simulink model "talos_navigation"  (R2023a)
settings: Solver=FixedStepDiscrete  StartTime=0.0  StopTime=10.0  FixedStep=1/1000.0  RelTol=1e-3  EnableMultiTasking=on
undefined symbols (not defined in the file): accel, child_frame_id, child_frame_id_SL_Info, data, data_SL_Info, header, layout, transform, transforms, transforms_SL_Info
libraries: ros2lib x187, simulink x9, sharedTrackingLibrary x1
(part 3 of 3)

== system talos_navigation/Parameters/estimator/process_noise_diag ==
  element_0 : ros2lib/Get Parameter  ParameterName=navigation__estimator__process_noise_diag_0  ParameterType=double  ParameterMaxArrayLength=16  ParameterInitialValue=5e-05  SampleTime=1/10.0  ModelName=ros2lib  BlockId=ParamGet_ros2lib_196
  element_1 : ros2lib/Get Parameter  ParameterName=navigation__estimator__process_noise_diag_1  ParameterType=double  ParameterMaxArrayLength=16  ParameterInitialValue=5e-05  SampleTime=1/10.0  ModelName=ros2lib  BlockId=ParamGet_ros2lib_196
  element_10 : ros2lib/Get Parameter  ParameterName=navigation__estimator__process_noise_diag_10  ParameterType=double  ParameterMaxArrayLength=16  ParameterInitialValue=0.0003  SampleTime=1/10.0  ModelName=ros2lib  BlockId=ParamGet_ros2lib_196
  element_11 : ros2lib/Get Parameter  ParameterName=navigation__estimator__process_noise_diag_11  ParameterType=double  ParameterMaxArrayLength=16  ParameterInitialValue=0.0003  SampleTime=1/10.0  ModelName=ros2lib  BlockId=ParamGet_ros2lib_196
  element_12 : ros2lib/Get Parameter  ParameterName=navigation__estimator__process_noise_diag_12  ParameterType=double  ParameterMaxArrayLength=16  ParameterInitialValue=0.0006  SampleTime=1/10.0  ModelName=ros2lib  BlockId=ParamGet_ros2lib_196
  element_13 : ros2lib/Get Parameter  ParameterName=navigation__estimator__process_noise_diag_13  ParameterType=double  ParameterMaxArrayLength=16  ParameterInitialValue=0.0003  SampleTime=1/10.0  ModelName=ros2lib  BlockId=ParamGet_ros2lib_196
  element_14 : ros2lib/Get Parameter  ParameterName=navigation__estimator__process_noise_diag_14  ParameterType=double  ParameterMaxArrayLength=16  ParameterInitialValue=0.0003  SampleTime=1/10.0  ModelName=ros2lib  BlockId=ParamGet_ros2lib_196
  element_15 : ros2lib/Get Parameter  ParameterName=navigation__estimator__process_noise_diag_15  ParameterType=double  ParameterMaxArrayLength=16  ParameterInitialValue=0.00045  SampleTime=1/10.0  ModelName=ros2lib  BlockId=ParamGet_ros2lib_196
  element_2 : ros2lib/Get Parameter  ParameterName=navigation__estimator__process_noise_diag_2  ParameterType=double  ParameterMaxArrayLength=16  ParameterInitialValue=6e-05  SampleTime=1/10.0  ModelName=ros2lib  BlockId=ParamGet_ros2lib_196
  element_3 : ros2lib/Get Parameter  ParameterName=navigation__estimator__process_noise_diag_3  ParameterType=double  ParameterMaxArrayLength=16  ParameterInitialValue=3e-05  SampleTime=1/10.0  ModelName=ros2lib  BlockId=ParamGet_ros2lib_196
  element_4 : ros2lib/Get Parameter  ParameterName=navigation__estimator__process_noise_diag_4  ParameterType=double  ParameterMaxArrayLength=16  ParameterInitialValue=3e-05  SampleTime=1/10.0  ModelName=ros2lib  BlockId=ParamGet_ros2lib_196
  element_5 : ros2lib/Get Parameter  ParameterName=navigation__estimator__process_noise_diag_5  ParameterType=double  ParameterMaxArrayLength=16  ParameterInitialValue=6e-05  SampleTime=1/10.0  ModelName=ros2lib  BlockId=ParamGet_ros2lib_196
  element_6 : ros2lib/Get Parameter  ParameterName=navigation__estimator__process_noise_diag_6  ParameterType=double  ParameterMaxArrayLength=16  ParameterInitialValue=1e-06  SampleTime=1/10.0  ModelName=ros2lib  BlockId=ParamGet_ros2lib_196
  element_7 : ros2lib/Get Parameter  ParameterName=navigation__estimator__process_noise_diag_7  ParameterType=double  ParameterMaxArrayLength=16  ParameterInitialValue=0.0025  SampleTime=1/10.0  ModelName=ros2lib  BlockId=ParamGet_ros2lib_196
  element_8 : ros2lib/Get Parameter  ParameterName=navigation__estimator__process_noise_diag_8  ParameterType=double  ParameterMaxArrayLength=16  ParameterInitialValue=0.0025  SampleTime=1/10.0  ModelName=ros2lib  BlockId=ParamGet_ros2lib_196
  element_9 : ros2lib/Get Parameter  ParameterName=navigation__estimator__process_noise_diag_9  ParameterType=double  ParameterMaxArrayLength=16  ParameterInitialValue=0.004  SampleTime=1/10.0  ModelName=ros2lib  BlockId=ParamGet_ros2lib_196
  elements : Concatenate  NumInputs=16
  value : Outport
  wires:
  element_0/1 -> elements/1
  element_1/1 -> elements/2
  element_2/1 -> elements/3
  element_3/1 -> elements/4
  element_4/1 -> elements/5
  element_5/1 -> elements/6
  element_6/1 -> elements/7
  element_7/1 -> elements/8
  element_8/1 -> elements/9
  element_9/1 -> elements/10
  element_10/1 -> elements/11
  element_11/1 -> elements/12
  element_12/1 -> elements/13
  element_13/1 -> elements/14
  element_14/1 -> elements/15
  element_15/1 -> elements/16
  elements/1 -> value/1

== system talos_navigation/Parameters/estimator/reset_covariance_diag ==
  element_0 : ros2lib/Get Parameter  ParameterName=navigation__estimator__reset_covariance_diag_0  ParameterType=double  ParameterMaxArrayLength=16  ParameterInitialValue=1  SampleTime=1/10.0  ModelName=ros2lib  BlockId=ParamGet_ros2lib_196
  element_1 : ros2lib/Get Parameter  ParameterName=navigation__estimator__reset_covariance_diag_1  ParameterType=double  ParameterMaxArrayLength=16  ParameterInitialValue=1  SampleTime=1/10.0  ModelName=ros2lib  BlockId=ParamGet_ros2lib_196
  element_10 : ros2lib/Get Parameter  ParameterName=navigation__estimator__reset_covariance_diag_10  ParameterType=double  ParameterMaxArrayLength=16  ParameterInitialValue=0.05  SampleTime=1/10.0  ModelName=ros2lib  BlockId=ParamGet_ros2lib_196
  element_11 : ros2lib/Get Parameter  ParameterName=navigation__estimator__reset_covariance_diag_11  ParameterType=double  ParameterMaxArrayLength=16  ParameterInitialValue=0.05  SampleTime=1/10.0  ModelName=ros2lib  BlockId=ParamGet_ros2lib_196
  element_12 : ros2lib/Get Parameter  ParameterName=navigation__estimator__reset_covariance_diag_12  ParameterType=double  ParameterMaxArrayLength=16  ParameterInitialValue=0.05  SampleTime=1/10.0  ModelName=ros2lib  BlockId=ParamGet_ros2lib_196
  element_13 : ros2lib/Get Parameter  ParameterName=navigation__estimator__reset_covariance_diag_13  ParameterType=double  ParameterMaxArrayLength=16  ParameterInitialValue=0.5  SampleTime=1/10.0  ModelName=ros2lib  BlockId=ParamGet_ros2lib_196
  element_14 : ros2lib/Get Parameter  ParameterName=navigation__estimator__reset_covariance_diag_14  ParameterType=double  ParameterMaxArrayLength=16  ParameterInitialValue=0.5  SampleTime=1/10.0  ModelName=ros2lib  BlockId=ParamGet_ros2lib_196
  element_15 : ros2lib/Get Parameter  ParameterName=navigation__estimator__reset_covariance_diag_15  ParameterType=double  ParameterMaxArrayLength=16  ParameterInitialValue=0.5  SampleTime=1/10.0  ModelName=ros2lib  BlockId=ParamGet_ros2lib_196
  element_2 : ros2lib/Get Parameter  ParameterName=navigation__estimator__reset_covariance_diag_2  ParameterType=double  ParameterMaxArrayLength=16  ParameterInitialValue=0.25  SampleTime=1/10.0  ModelName=ros2lib  BlockId=ParamGet_ros2lib_196
  element_3 : ros2lib/Get Parameter  ParameterName=navigation__estimator__reset_covariance_diag_3  ParameterType=double  ParameterMaxArrayLength=16  ParameterInitialValue=0  SampleTime=1/10.0  ModelName=ros2lib  BlockId=ParamGet_ros2lib_196
  element_4 : ros2lib/Get Parameter  ParameterName=navigation__estimator__reset_covariance_diag_4  ParameterType=double  ParameterMaxArrayLength=16  ParameterInitialValue=0.00025  SampleTime=1/10.0  ModelName=ros2lib  BlockId=ParamGet_ros2lib_196
  element_5 : ros2lib/Get Parameter  ParameterName=navigation__estimator__reset_covariance_diag_5  ParameterType=double  ParameterMaxArrayLength=16  ParameterInitialValue=0.00025  SampleTime=1/10.0  ModelName=ros2lib  BlockId=ParamGet_ros2lib_196
  element_6 : ros2lib/Get Parameter  ParameterName=navigation__estimator__reset_covariance_diag_6  ParameterType=double  ParameterMaxArrayLength=16  ParameterInitialValue=0.00025  SampleTime=1/10.0  ModelName=ros2lib  BlockId=ParamGet_ros2lib_196
  element_7 : ros2lib/Get Parameter  ParameterName=navigation__estimator__reset_covariance_diag_7  ParameterType=double  ParameterMaxArrayLength=16  ParameterInitialValue=0.25  SampleTime=1/10.0  ModelName=ros2lib  BlockId=ParamGet_ros2lib_196
  element_8 : ros2lib/Get Parameter  ParameterName=navigation__estimator__reset_covariance_diag_8  ParameterType=double  ParameterMaxArrayLength=16  ParameterInitialValue=0.25  SampleTime=1/10.0  ModelName=ros2lib  BlockId=ParamGet_ros2lib_196
  element_9 : ros2lib/Get Parameter  ParameterName=navigation__estimator__reset_covariance_diag_9  ParameterType=double  ParameterMaxArrayLength=16  ParameterInitialValue=0.25  SampleTime=1/10.0  ModelName=ros2lib  BlockId=ParamGet_ros2lib_196
  elements : Concatenate  NumInputs=16
  value : Outport
  wires:
  element_0/1 -> elements/1
  element_1/1 -> elements/2
  element_2/1 -> elements/3
  element_3/1 -> elements/4
  element_4/1 -> elements/5
  element_5/1 -> elements/6
  element_6/1 -> elements/7
  element_7/1 -> elements/8
  element_8/1 -> elements/9
  element_9/1 -> elements/10
  element_10/1 -> elements/11
  element_11/1 -> elements/12
  element_12/1 -> elements/13
  element_13/1 -> elements/14
  element_14/1 -> elements/15
  element_15/1 -> elements/16
  elements/1 -> value/1

== system talos_navigation/Parameters/gates/gate_consistency_stddev ==
  element_0 : ros2lib/Get Parameter  ParameterName=navigation__gates__gate_consistency_stddev_0  ParameterType=double  ParameterMaxArrayLength=16  ParameterInitialValue=0.01  SampleTime=1/10.0  ModelName=ros2lib  BlockId=ParamGet_ros2lib_196
  element_1 : ros2lib/Get Parameter  ParameterName=navigation__gates__gate_consistency_stddev_1  ParameterType=double  ParameterMaxArrayLength=16  ParameterInitialValue=0.02  SampleTime=1/10.0  ModelName=ros2lib  BlockId=ParamGet_ros2lib_196
  element_2 : ros2lib/Get Parameter  ParameterName=navigation__gates__gate_consistency_stddev_2  ParameterType=double  ParameterMaxArrayLength=16  ParameterInitialValue=0.05  SampleTime=1/10.0  ModelName=ros2lib  BlockId=ParamGet_ros2lib_196
  element_3 : ros2lib/Get Parameter  ParameterName=navigation__gates__gate_consistency_stddev_3  ParameterType=double  ParameterMaxArrayLength=16  ParameterInitialValue=0.02  SampleTime=1/10.0  ModelName=ros2lib  BlockId=ParamGet_ros2lib_196
  elements : Concatenate  NumInputs=4
  value : Outport
  wires:
  element_0/1 -> elements/1
  element_1/1 -> elements/2
  element_2/1 -> elements/3
  element_3/1 -> elements/4
  elements/1 -> value/1

== system talos_navigation/Parameters/mounts/depth_rotation ==
  element_0 : ros2lib/Get Parameter  ParameterName=navigation__mounts__depth_rotation_0  ParameterType=double  ParameterMaxArrayLength=16  ParameterInitialValue=1  SampleTime=1/10.0  ModelName=ros2lib  BlockId=ParamGet_ros2lib_196
  element_1 : ros2lib/Get Parameter  ParameterName=navigation__mounts__depth_rotation_1  ParameterType=double  ParameterMaxArrayLength=16  ParameterInitialValue=0  SampleTime=1/10.0  ModelName=ros2lib  BlockId=ParamGet_ros2lib_196
  element_2 : ros2lib/Get Parameter  ParameterName=navigation__mounts__depth_rotation_2  ParameterType=double  ParameterMaxArrayLength=16  ParameterInitialValue=0  SampleTime=1/10.0  ModelName=ros2lib  BlockId=ParamGet_ros2lib_196
  element_3 : ros2lib/Get Parameter  ParameterName=navigation__mounts__depth_rotation_3  ParameterType=double  ParameterMaxArrayLength=16  ParameterInitialValue=0  SampleTime=1/10.0  ModelName=ros2lib  BlockId=ParamGet_ros2lib_196
  elements : Concatenate  NumInputs=4
  value : Outport
  wires:
  element_0/1 -> elements/1
  element_1/1 -> elements/2
  element_2/1 -> elements/3
  element_3/1 -> elements/4
  elements/1 -> value/1

== system talos_navigation/Parameters/mounts/depth_translation ==
  element_0 : ros2lib/Get Parameter  ParameterName=navigation__mounts__depth_translation_0  ParameterType=double  ParameterMaxArrayLength=16  ParameterInitialValue=0  SampleTime=1/10.0  ModelName=ros2lib  BlockId=ParamGet_ros2lib_196
  element_1 : ros2lib/Get Parameter  ParameterName=navigation__mounts__depth_translation_1  ParameterType=double  ParameterMaxArrayLength=16  ParameterInitialValue=0  SampleTime=1/10.0  ModelName=ros2lib  BlockId=ParamGet_ros2lib_196
  element_2 : ros2lib/Get Parameter  ParameterName=navigation__mounts__depth_translation_2  ParameterType=double  ParameterMaxArrayLength=16  ParameterInitialValue=0  SampleTime=1/10.0  ModelName=ros2lib  BlockId=ParamGet_ros2lib_196
  elements : Concatenate  NumInputs=3
  value : Outport
  wires:
  element_0/1 -> elements/1
  element_1/1 -> elements/2
  element_2/1 -> elements/3
  elements/1 -> value/1

== system talos_navigation/Parameters/mounts/dvl_rotation ==
  element_0 : ros2lib/Get Parameter  ParameterName=navigation__mounts__dvl_rotation_0  ParameterType=double  ParameterMaxArrayLength=16  ParameterInitialValue=1  SampleTime=1/10.0  ModelName=ros2lib  BlockId=ParamGet_ros2lib_196
  element_1 : ros2lib/Get Parameter  ParameterName=navigation__mounts__dvl_rotation_1  ParameterType=double  ParameterMaxArrayLength=16  ParameterInitialValue=0  SampleTime=1/10.0  ModelName=ros2lib  BlockId=ParamGet_ros2lib_196
  element_2 : ros2lib/Get Parameter  ParameterName=navigation__mounts__dvl_rotation_2  ParameterType=double  ParameterMaxArrayLength=16  ParameterInitialValue=0  SampleTime=1/10.0  ModelName=ros2lib  BlockId=ParamGet_ros2lib_196
  element_3 : ros2lib/Get Parameter  ParameterName=navigation__mounts__dvl_rotation_3  ParameterType=double  ParameterMaxArrayLength=16  ParameterInitialValue=0  SampleTime=1/10.0  ModelName=ros2lib  BlockId=ParamGet_ros2lib_196
  elements : Concatenate  NumInputs=4
  value : Outport
  wires:
  element_0/1 -> elements/1
  element_1/1 -> elements/2
  element_2/1 -> elements/3
  element_3/1 -> elements/4
  elements/1 -> value/1

== system talos_navigation/Parameters/mounts/dvl_translation ==
  element_0 : ros2lib/Get Parameter  ParameterName=navigation__mounts__dvl_translation_0  ParameterType=double  ParameterMaxArrayLength=16  ParameterInitialValue=0  SampleTime=1/10.0  ModelName=ros2lib  BlockId=ParamGet_ros2lib_196
  element_1 : ros2lib/Get Parameter  ParameterName=navigation__mounts__dvl_translation_1  ParameterType=double  ParameterMaxArrayLength=16  ParameterInitialValue=0  SampleTime=1/10.0  ModelName=ros2lib  BlockId=ParamGet_ros2lib_196
  element_2 : ros2lib/Get Parameter  ParameterName=navigation__mounts__dvl_translation_2  ParameterType=double  ParameterMaxArrayLength=16  ParameterInitialValue=0  SampleTime=1/10.0  ModelName=ros2lib  BlockId=ParamGet_ros2lib_196
  elements : Concatenate  NumInputs=3
  value : Outport
  wires:
  element_0/1 -> elements/1
  element_1/1 -> elements/2
  element_2/1 -> elements/3
  elements/1 -> value/1

== system talos_navigation/Parameters/mounts/fog_rotation ==
  element_0 : ros2lib/Get Parameter  ParameterName=navigation__mounts__fog_rotation_0  ParameterType=double  ParameterMaxArrayLength=16  ParameterInitialValue=1  SampleTime=1/10.0  ModelName=ros2lib  BlockId=ParamGet_ros2lib_196
  element_1 : ros2lib/Get Parameter  ParameterName=navigation__mounts__fog_rotation_1  ParameterType=double  ParameterMaxArrayLength=16  ParameterInitialValue=0  SampleTime=1/10.0  ModelName=ros2lib  BlockId=ParamGet_ros2lib_196
  element_2 : ros2lib/Get Parameter  ParameterName=navigation__mounts__fog_rotation_2  ParameterType=double  ParameterMaxArrayLength=16  ParameterInitialValue=0  SampleTime=1/10.0  ModelName=ros2lib  BlockId=ParamGet_ros2lib_196
  element_3 : ros2lib/Get Parameter  ParameterName=navigation__mounts__fog_rotation_3  ParameterType=double  ParameterMaxArrayLength=16  ParameterInitialValue=0  SampleTime=1/10.0  ModelName=ros2lib  BlockId=ParamGet_ros2lib_196
  elements : Concatenate  NumInputs=4
  value : Outport
  wires:
  element_0/1 -> elements/1
  element_1/1 -> elements/2
  element_2/1 -> elements/3
  element_3/1 -> elements/4
  elements/1 -> value/1

== system talos_navigation/Parameters/mounts/fog_translation ==
  element_0 : ros2lib/Get Parameter  ParameterName=navigation__mounts__fog_translation_0  ParameterType=double  ParameterMaxArrayLength=16  ParameterInitialValue=0  SampleTime=1/10.0  ModelName=ros2lib  BlockId=ParamGet_ros2lib_196
  element_1 : ros2lib/Get Parameter  ParameterName=navigation__mounts__fog_translation_1  ParameterType=double  ParameterMaxArrayLength=16  ParameterInitialValue=0  SampleTime=1/10.0  ModelName=ros2lib  BlockId=ParamGet_ros2lib_196
  element_2 : ros2lib/Get Parameter  ParameterName=navigation__mounts__fog_translation_2  ParameterType=double  ParameterMaxArrayLength=16  ParameterInitialValue=0  SampleTime=1/10.0  ModelName=ros2lib  BlockId=ParamGet_ros2lib_196
  elements : Concatenate  NumInputs=3
  value : Outport
  wires:
  element_0/1 -> elements/1
  element_1/1 -> elements/2
  element_2/1 -> elements/3
  elements/1 -> value/1

== system talos_navigation/Parameters/mounts/imu_rotation ==
  element_0 : ros2lib/Get Parameter  ParameterName=navigation__mounts__imu_rotation_0  ParameterType=double  ParameterMaxArrayLength=16  ParameterInitialValue=1  SampleTime=1/10.0  ModelName=ros2lib  BlockId=ParamGet_ros2lib_196
  element_1 : ros2lib/Get Parameter  ParameterName=navigation__mounts__imu_rotation_1  ParameterType=double  ParameterMaxArrayLength=16  ParameterInitialValue=0  SampleTime=1/10.0  ModelName=ros2lib  BlockId=ParamGet_ros2lib_196
  element_2 : ros2lib/Get Parameter  ParameterName=navigation__mounts__imu_rotation_2  ParameterType=double  ParameterMaxArrayLength=16  ParameterInitialValue=0  SampleTime=1/10.0  ModelName=ros2lib  BlockId=ParamGet_ros2lib_196
  element_3 : ros2lib/Get Parameter  ParameterName=navigation__mounts__imu_rotation_3  ParameterType=double  ParameterMaxArrayLength=16  ParameterInitialValue=0  SampleTime=1/10.0  ModelName=ros2lib  BlockId=ParamGet_ros2lib_196
  elements : Concatenate  NumInputs=4
  value : Outport
  wires:
  element_0/1 -> elements/1
  element_1/1 -> elements/2
  element_2/1 -> elements/3
  element_3/1 -> elements/4
  elements/1 -> value/1

== system talos_navigation/Parameters/mounts/imu_translation ==
  element_0 : ros2lib/Get Parameter  ParameterName=navigation__mounts__imu_translation_0  ParameterType=double  ParameterMaxArrayLength=16  ParameterInitialValue=0  SampleTime=1/10.0  ModelName=ros2lib  BlockId=ParamGet_ros2lib_196
  element_1 : ros2lib/Get Parameter  ParameterName=navigation__mounts__imu_translation_1  ParameterType=double  ParameterMaxArrayLength=16  ParameterInitialValue=0  SampleTime=1/10.0  ModelName=ros2lib  BlockId=ParamGet_ros2lib_196
  element_2 : ros2lib/Get Parameter  ParameterName=navigation__mounts__imu_translation_2  ParameterType=double  ParameterMaxArrayLength=16  ParameterInitialValue=0  SampleTime=1/10.0  ModelName=ros2lib  BlockId=ParamGet_ros2lib_196
  elements : Concatenate  NumInputs=3
  value : Outport
  wires:
  element_0/1 -> elements/1
  element_1/1 -> elements/2
  element_2/1 -> elements/3
  elements/1 -> value/1

== system talos_navigation/Parameters/sensor_axes/dvl_axis_multiplier ==
  element_0 : ros2lib/Get Parameter  ParameterName=navigation__sensor_axes__dvl_axis_multiplier_0  ParameterType=double  ParameterMaxArrayLength=16  ParameterInitialValue=1  SampleTime=1/10.0  ModelName=ros2lib  BlockId=ParamGet_ros2lib_196
  element_1 : ros2lib/Get Parameter  ParameterName=navigation__sensor_axes__dvl_axis_multiplier_1  ParameterType=double  ParameterMaxArrayLength=16  ParameterInitialValue=1  SampleTime=1/10.0  ModelName=ros2lib  BlockId=ParamGet_ros2lib_196
  element_2 : ros2lib/Get Parameter  ParameterName=navigation__sensor_axes__dvl_axis_multiplier_2  ParameterType=double  ParameterMaxArrayLength=16  ParameterInitialValue=1  SampleTime=1/10.0  ModelName=ros2lib  BlockId=ParamGet_ros2lib_196
  elements : Concatenate  NumInputs=3
  value : Outport
  wires:
  element_0/1 -> elements/1
  element_1/1 -> elements/2
  element_2/1 -> elements/3
  elements/1 -> value/1

== system talos_navigation/Parameters/sensor_axes/fog_axis_multiplier ==
  element_0 : ros2lib/Get Parameter  ParameterName=navigation__sensor_axes__fog_axis_multiplier_0  ParameterType=double  ParameterMaxArrayLength=16  ParameterInitialValue=1  SampleTime=1/10.0  ModelName=ros2lib  BlockId=ParamGet_ros2lib_196
  element_1 : ros2lib/Get Parameter  ParameterName=navigation__sensor_axes__fog_axis_multiplier_1  ParameterType=double  ParameterMaxArrayLength=16  ParameterInitialValue=1  SampleTime=1/10.0  ModelName=ros2lib  BlockId=ParamGet_ros2lib_196
  element_2 : ros2lib/Get Parameter  ParameterName=navigation__sensor_axes__fog_axis_multiplier_2  ParameterType=double  ParameterMaxArrayLength=16  ParameterInitialValue=1  SampleTime=1/10.0  ModelName=ros2lib  BlockId=ParamGet_ros2lib_196
  elements : Concatenate  NumInputs=3
  value : Outport
  wires:
  element_0/1 -> elements/1
  element_1/1 -> elements/2
  element_2/1 -> elements/3
  elements/1 -> value/1

== system talos_navigation/Parameters/sensor_axes/imu_acceleration_axis_multiplier ==
  element_0 : ros2lib/Get Parameter  ParameterName=navigation__sensor_axes__imu_acceleration_axis_multiplier_0  ParameterType=double  ParameterMaxArrayLength=16  ParameterInitialValue=1  SampleTime=1/10.0  ModelName=ros2lib  BlockId=ParamGet_ros2lib_196
  element_1 : ros2lib/Get Parameter  ParameterName=navigation__sensor_axes__imu_acceleration_axis_multiplier_1  ParameterType=double  ParameterMaxArrayLength=16  ParameterInitialValue=1  SampleTime=1/10.0  ModelName=ros2lib  BlockId=ParamGet_ros2lib_196
  element_2 : ros2lib/Get Parameter  ParameterName=navigation__sensor_axes__imu_acceleration_axis_multiplier_2  ParameterType=double  ParameterMaxArrayLength=16  ParameterInitialValue=1  SampleTime=1/10.0  ModelName=ros2lib  BlockId=ParamGet_ros2lib_196
  elements : Concatenate  NumInputs=3
  value : Outport
  wires:
  element_0/1 -> elements/1
  element_1/1 -> elements/2
  element_2/1 -> elements/3
  elements/1 -> value/1

== system talos_navigation/Parameters/sensor_axes/imu_angular_velocity_axis_multiplier ==
  element_0 : ros2lib/Get Parameter  ParameterName=navigation__sensor_axes__imu_angular_velocity_axis_multiplier_0  ParameterType=double  ParameterMaxArrayLength=16  ParameterInitialValue=1  SampleTime=1/10.0  ModelName=ros2lib  BlockId=ParamGet_ros2lib_196
  element_1 : ros2lib/Get Parameter  ParameterName=navigation__sensor_axes__imu_angular_velocity_axis_multiplier_1  ParameterType=double  ParameterMaxArrayLength=16  ParameterInitialValue=1  SampleTime=1/10.0  ModelName=ros2lib  BlockId=ParamGet_ros2lib_196
  element_2 : ros2lib/Get Parameter  ParameterName=navigation__sensor_axes__imu_angular_velocity_axis_multiplier_2  ParameterType=double  ParameterMaxArrayLength=16  ParameterInitialValue=1  SampleTime=1/10.0  ModelName=ros2lib  BlockId=ParamGet_ros2lib_196
  elements : Concatenate  NumInputs=3
  value : Outport
  wires:
  element_0/1 -> elements/1
  element_1/1 -> elements/2
  element_2/1 -> elements/3
  elements/1 -> value/1

== system talos_navigation/Parameters/sensor_axes/imu_orientation_axis_multiplier ==
  element_0 : ros2lib/Get Parameter  ParameterName=navigation__sensor_axes__imu_orientation_axis_multiplier_0  ParameterType=double  ParameterMaxArrayLength=16  ParameterInitialValue=1  SampleTime=1/10.0  ModelName=ros2lib  BlockId=ParamGet_ros2lib_196
  element_1 : ros2lib/Get Parameter  ParameterName=navigation__sensor_axes__imu_orientation_axis_multiplier_1  ParameterType=double  ParameterMaxArrayLength=16  ParameterInitialValue=1  SampleTime=1/10.0  ModelName=ros2lib  BlockId=ParamGet_ros2lib_196
  element_2 : ros2lib/Get Parameter  ParameterName=navigation__sensor_axes__imu_orientation_axis_multiplier_2  ParameterType=double  ParameterMaxArrayLength=16  ParameterInitialValue=1  SampleTime=1/10.0  ModelName=ros2lib  BlockId=ParamGet_ros2lib_196
  elements : Concatenate  NumInputs=3
  value : Outport
  wires:
  element_0/1 -> elements/1
  element_1/1 -> elements/2
  element_2/1 -> elements/3
  elements/1 -> value/1

== system talos_navigation/Parameters/timing/sensor_timeouts ==
  element_0 : ros2lib/Get Parameter  ParameterName=navigation__timing__sensor_timeouts_0  ParameterType=double  ParameterMaxArrayLength=16  ParameterInitialValue=0.25  SampleTime=1/10.0  ModelName=ros2lib  BlockId=ParamGet_ros2lib_196
  element_1 : ros2lib/Get Parameter  ParameterName=navigation__timing__sensor_timeouts_1  ParameterType=double  ParameterMaxArrayLength=16  ParameterInitialValue=0.25  SampleTime=1/10.0  ModelName=ros2lib  BlockId=ParamGet_ros2lib_196
  element_2 : ros2lib/Get Parameter  ParameterName=navigation__timing__sensor_timeouts_2  ParameterType=double  ParameterMaxArrayLength=16  ParameterInitialValue=0.5  SampleTime=1/10.0  ModelName=ros2lib  BlockId=ParamGet_ros2lib_196
  element_3 : ros2lib/Get Parameter  ParameterName=navigation__timing__sensor_timeouts_3  ParameterType=double  ParameterMaxArrayLength=16  ParameterInitialValue=0.5  SampleTime=1/10.0  ModelName=ros2lib  BlockId=ParamGet_ros2lib_196
  elements : Concatenate  NumInputs=4
  value : Outport
  wires:
  element_0/1 -> elements/1
  element_1/1 -> elements/2
  element_2/1 -> elements/3
  element_3/1 -> elements/4
  elements/1 -> value/1

== system talos_navigation/Publish_System/Acceleration/fill_publish ==
  msg : Inport
  Enable : EnablePort
  Publish : ros2lib/Publish  topicSource=Select from ROS network  topic=accel/filtered  messageType=geometry_msgs/AccelWithCovarianceStamped  QOSHistory=Keep last  QOSDepth=1  QOSReliability=Reliable  QOSDurability=Volatile
  wires:
  msg/1 -> Publish/1

== system talos_navigation/Publish_System/Diagnostics/part_0_publish ==
  msg : Inport
  Enable : EnablePort
  Publish : ros2lib/Publish  topicSource=Select from ROS network  topic=navigation/diagnostics  messageType=std_msgs/Float64MultiArray  QOSHistory=Keep last  QOSDepth=1  QOSReliability=Reliable  QOSDurability=Volatile
  wires:
  msg/1 -> Publish/1

== system talos_navigation/Publish_System/Diagnostics/part_1_publish ==
  msg : Inport
  Enable : EnablePort
  Publish : ros2lib/Publish  topicSource=Select from ROS network  topic=navigation/diagnostics  messageType=std_msgs/Float64MultiArray  QOSHistory=Keep last  QOSDepth=1  QOSReliability=Reliable  QOSDurability=Volatile
  wires:
  msg/1 -> Publish/1

== system talos_navigation/Publish_System/Odometry/fill_publish ==
  msg : Inport
  Enable : EnablePort
  Publish : ros2lib/Publish  topicSource=Select from ROS network  topic=odometry/filtered  messageType=nav_msgs/Odometry  QOSHistory=Keep last  QOSDepth=1  QOSReliability=Reliable  QOSDurability=Volatile
  wires:
  msg/1 -> Publish/1

== system talos_navigation/Publish_System/TF/tf_message_publish ==
  msg : Inport
  Enable : EnablePort
  Publish : ros2lib/Publish  topicSource=Select from ROS network  topic=/tf  messageType=tf2_msgs/TFMessage  QOSHistory=Keep last  QOSDepth=1  QOSReliability=Reliable  QOSDurability=Volatile
  wires:
  msg/1 -> Publish/1

== matlab function talos_navigation/Measurement_Intake/FOG/Frame_Kind ==
  data: frame_id input; frame output; n input; base input; mount input
function frame = kind(frame_id, n, base, mount)
frame = talos_nav_frame_kind(frame_id, n, base, mount);

== matlab function talos_navigation/Measurement_Intake/IMU/Frame_Kind ==
  data: frame_id input; frame output; n input; base input; mount input
function frame = kind(frame_id, n, base, mount)
frame = talos_nav_frame_kind(frame_id, n, base, mount);

== matlab function talos_navigation/Measurement_Intake/DVL/Frame_Kind ==
  data: frame_id input; frame output; n input; base input; mount input
function frame = kind(frame_id, n, base, mount)
frame = talos_nav_frame_kind(frame_id, n, base, mount);

== matlab function talos_navigation/Measurement_Intake/Depth/Frame_Kind ==
  data: frame_id input; frame output; n input; base input; world input; depth_frame input; mount output
function [frame, mount] = kind(frame_id, n, base, world, depth_frame)
% world kind, and whether the sample is in the overseer's depth_frame
frame = talos_nav_world_kind(frame_id, n, base, world);
mount = talos_nav_frame_match(frame_id, n, depth_frame);

== matlab function talos_navigation/Measurement_Intake/Depth/Depth_Mount/Rotation_Matrix ==
  data: q input; R output
function R = rotation(q)
% body to world matrix of the quaternion [w; x; y; z]
R = talos_nav_rotation(q);

== matlab function talos_navigation/Measurement_Intake/Set_Pose/Frame_Kind ==
  data: frame_id input; frame output; n input; base input; world input
function frame = kind(frame_id, n, base, world)
frame = talos_nav_world_kind(frame_id, n, base, world);

== matlab function talos_navigation/Measurement_Intake/Input_Ring ==
  data: raw input Bus: talos_nav_raw; ring output size=1955; arrival input; taken input
function ring = input_ring(raw, arrival, taken)
% see talos_nav_ring_write
ring = talos_nav_ring_write(raw, arrival, taken);
end

== matlab function talos_navigation/Estimator/Fusion ==
  data: param_bus input Bus: talos_nav_params; pub output boolean size=1; ring input; now input; started input; publish input; diagnostics input; x output double size=19; P output double size=[19 19]; pose_cov output double size=[6 6]; d output double size=162; taken output double size=1
function [pub, x, P, pose_cov, d, taken] = fusion(param_bus, ring, now, started, publish, diagnostics)
% see talos_nav_fusion; the filter is the Extended Kalman Filter block
[pub, x, P, pose_cov, d, taken] = talos_nav_fusion(param_bus, ring, now, started, publish, diagnostics, @ekf);
end

function [x, P] = ekf(x, P, dt, Sq, sensor, y, R, ctx)
[x, P] = talos_nav_ekf(@step, x, P, dt, Sq, sensor, y, R, ctx);
end

function [x, P] = step(mode, dt, Sq, x0, sensor, y, R, ctx)
[x, P] = talos_nav_ekf_step(mode, dt, Sq, x0, sensor, y, R, ctx);
end
